simulink model "bicycle_trailer_trailer"  (R2025b)
settings: Solver=ode45  StartTime=0.0  StopTime=60  MaxStep=0.01  RelTol=1e-3
settings Model: Creator=Andrea  LastModifiedBy=Andrea

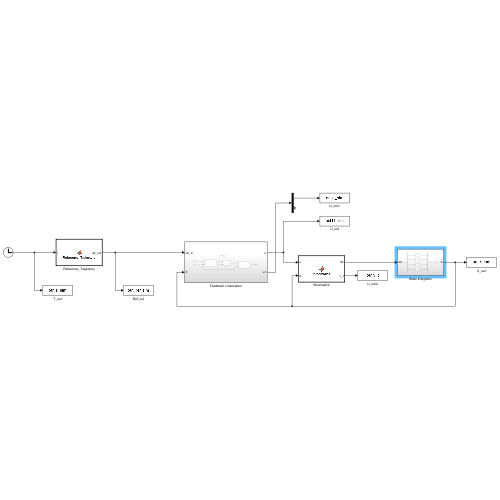
[thumbnail: Simulink's stored preview of the top-level diagram]
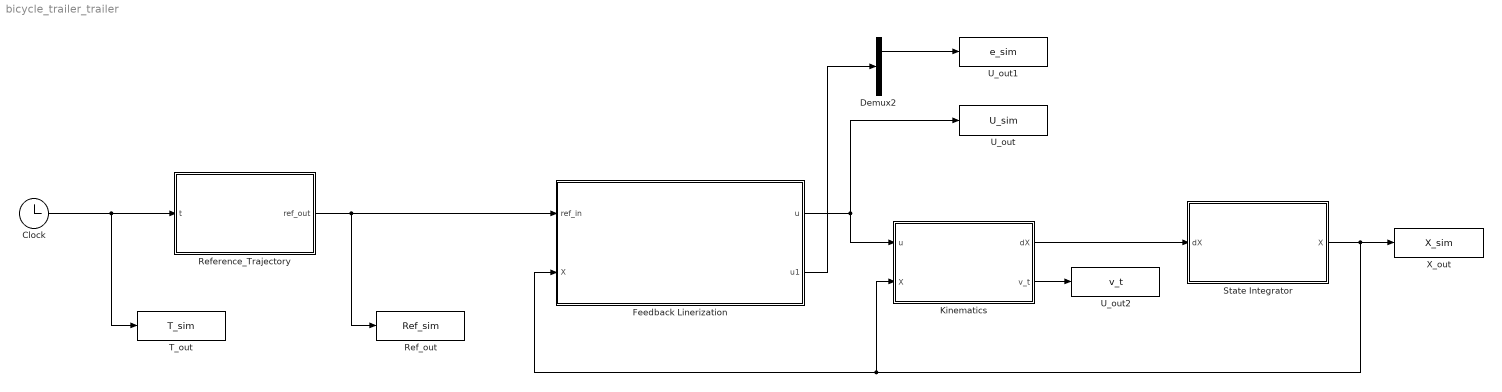
== system bicycle_trailer_trailer ==
  Clock : Clock
  Demux2 : Demux  Outputs=2
  Feedback Linerization : Subsystem
  Kinematics : MATLAB Function  TreatAsAtomicUnit=on
  Ref_out : ToWorkspace  VariableName=Ref_sim  SampleTime=-1
  Reference_Trajectory : MATLAB Function  TreatAsAtomicUnit=on
  State Integrator : Subsystem
  T_out : ToWorkspace  VariableName=T_sim  SampleTime=-1
  U_out : ToWorkspace  VariableName=U_sim  SampleTime=-1
  U_out1 : ToWorkspace  VariableName=e_sim  SampleTime=-1
  U_out2 : ToWorkspace  VariableName=v_t  SampleTime=-1
  X_out : ToWorkspace  VariableName=X_sim  SampleTime=-1
  wires:
  Clock/1 -> T_out/1, Reference_Trajectory/1(t)
  Reference_Trajectory/1(ref_out) -> Feedback Linerization/1(ref_in), Ref_out/1
  Feedback Linerization/1(u) -> Kinematics/1(u), U_out/1
  Demux2/1 -> U_out1/1
  Feedback Linerization/2(u1) -> Demux2/1
  Kinematics/2(v_t) -> U_out2/1
  Kinematics/1(dX) -> State Integrator/1(dX)
  State Integrator/1(X) -> Feedback Linerization/2(X), Kinematics/2(X), X_out/1

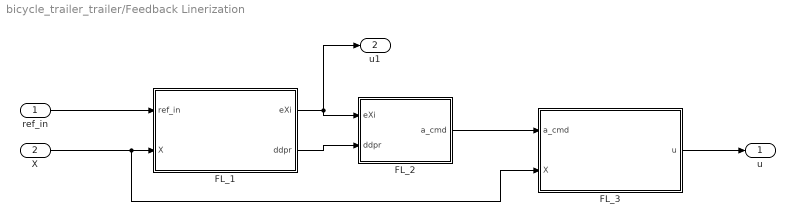
== system bicycle_trailer_trailer/Feedback Linerization ==
  ref_in : Inport
  X : Inport  Port=2
  FL_1 : MATLAB Function  TreatAsAtomicUnit=on
  FL_2 : MATLAB Function  TreatAsAtomicUnit=on
  FL_3 : MATLAB Function  TreatAsAtomicUnit=on
  u : Outport
  u1 : Outport  Port=2
  wires:
  FL_1/1(eXi) -> u1/1, FL_2/1(eXi)
  X/1 -> FL_3/2(X), FL_1/2(X)
  FL_2/1(a_cmd) -> FL_3/1(a_cmd)
  FL_3/1(u) -> u/1
  ref_in/1 -> FL_1/1(ref_in)
  FL_1/2(ddpr) -> FL_2/2(ddpr)

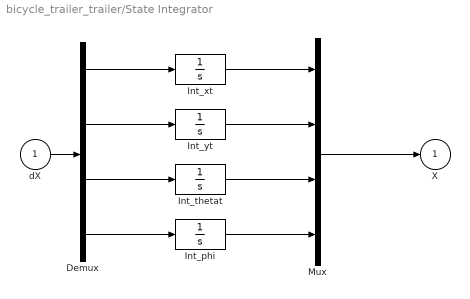
== system bicycle_trailer_trailer/State Integrator ==
  dX : Inport
  Demux : Demux
  Int_phi : Integrator  InitialCondition=0.08000000
  Int_thetat : Integrator  InitialCondition=1.67079633
  Int_xt : Integrator  InitialCondition=5
  Int_yt : Integrator  InitialCondition=8
  Mux : Mux
  X : Outport
  wires:
  dX/1 -> Demux/1
  Demux/1 -> Int_xt/1
  Int_xt/1 -> Mux/1
  Demux/2 -> Int_yt/1
  Int_yt/1 -> Mux/2
  Demux/3 -> Int_thetat/1
  Int_thetat/1 -> Mux/3
  Demux/4 -> Int_phi/1
  Int_phi/1 -> Mux/4
  Mux/1 -> X/1

== matlab function bicycle_trailer_trailer/Reference_Trajectory ==
  data: t input; ref_out output
function ref_out = Reference_Trajectory(t)
    ref_out = zeros(6,1);
    R=3.0000; w=0.2500; cx=0.0000; cy=0.0000;
    ref_out(1) =  cx + R*cos(w*t);
    ref_out(2) =  cy + R*sin(w*t);
    ref_out(3) = -R*w*sin(w*t);
    ref_out(4) =  R*w*cos(w*t);
    ref_out(5) = -R*w^2*cos(w*t);
    ref_out(6) = -R*w^2*sin(w*t);
end

== matlab function bicycle_trailer_trailer/Kinematics ==
  data: u input; dX output; X input; v_t output
function [dX,v_t] = Kinematics(u, X)
    dX = zeros(4,1);
    v_t = 0;
    L=1.0000; M=1.5000;
    v     = u(1);
    delta = u(2);
    theta_t = X(3);
    phi     = X(4);
    
    v_t = v * cos(phi);
    
    dX(1) = v_t * cos(theta_t);
    dX(2) = v_t * sin(theta_t);
    dX(3) = v_t * tan(phi) / M;
    dX(4) = v * tan(delta) / L - dX(3);
end

== matlab function bicycle_trailer_trailer/Feedback Linerization/FL_1 ==
  data: eXi output; ref_in input; X input; ddpr output
function [eXi,ddpr] = eXi(ref_in, X)
    d=0.55000;
    eXi = zeros(4,1);
    
    pr   = ref_in(1:2);
    dpr  = ref_in(3:4);
    ddpr = ref_in(5:6);
    
    x_t   = X(1); y_t = X(2); theta_t = X(3);
    
    % Punto virtuale sul rimorchio
    p = [x_t + d*cos(theta_t); y_t + d*sin(theta_t)];
    
    % Errore di tracking
    e  = p - pr;
    de = -dpr;
    eXi = [e;de];
end

== matlab function bicycle_trailer_trailer/Feedback Linerization/FL_2 ==
  data: eXi input; a_cmd output; ddpr input; K parameter
function a_cmd = LQR(eXi,ddpr,K)
    a_cmd = zeros(2,1);
    % LQR
    a_cmd = -K*eXi+ddpr;
end

== matlab function bicycle_trailer_trailer/Feedback Linerization/FL_3 ==
  data: a_cmd input; u output; X input

function u = Inversion(a_cmd, X)
    u = zeros(2,1);
    L=1.0000; M=1.5000; d=0.55000;
    kp_phi = 3.0;
    
    
    phi = X(4); theta_t = X(3);
    
    % Matrice di Decoupling
    A = [cos(theta_t), -d*sin(theta_t);
         sin(theta_t),  d*cos(theta_t)];
    
    % Inversione FL
    nu = zeros(2,1);
    if abs(d) > 1e-6
        nu = A \ a_cmd;
    else
        nu = pinv(J) * a_cmd;
    end
    
    % nu(1) = v_t,  nu(2) = v_t * tan(phi_des) / M
    v_t = nu(1);
    v_t = max(-3.0, min(3.0, v_t));
    
    % Angolo phi desiderato
    if abs(v_t) > 0.05
        phi_des = atan(nu(2) * M / v_t);
    else
        phi_des = 0;
    end
    phi_des = max(-0.7, min(0.7, phi_des));
    
    % Velocità fisica biciclo
    cphi = cos(phi);
    if abs(cphi) > 0.1
        v = v_t / cphi;
    else
        v = v_t * sign(cphi + 1e-9) / 0.1;
    end
    v = max(-3.5, min(3.5, v));
    
    %Curvatura rimorchio desiderata
    thetat_dot = v_t * tan(phi) / M;
    
    %Controllo phi con legge proporzionale
    phi_dot_des = kp_phi * (phi_des - phi);
    
    %Curvatura biciclo desiderata
    thetab_dot_des = phi_dot_des + thetat_dot;    
    
    % %Curvatura biciclo desiderata (senza il termine phi_dot_des)
    % thetab_dot_des = thetat_dot_des;
    
    % Angolo di sterzo
    if abs(v) > 0.05
        delta = atan(thetab_dot_des * L / v);
    else
        delta = atan(thetab_dot_des * L / 0.3) * sign(v + 1e-9);
    end
    delta = max(-0.6, min(0.6, delta));
    
    % Ingressi reali
    u(1) = v;
    u(2) = delta;
end
